simulink model "IEEE39_ClosedLoop_Native"  (R2025a)
settings: Solver=ode4  StartTime=0.0  StopTime=stopTime  FixedStep=dt  RelTol=1e-3
values from neighbouring files (symbols this model uses):
  dt = double(entry.step_s)    [run_fmu_cosim_sweep.m]    (also in run_ieee39_closed_loop.m; run_ieee39_native_closed_loop.m)
  loadStepTime = double(entry.load_step_s)    [run_ieee39_closed_loop.m]    (also in run_ieee39_native_closed_loop.m)
  stopTime = double(entry.stop_time_s)    [run_fmu_cosim_sweep.m]    (also in run_ieee39_closed_loop.m; run_ieee39_native_closed_loop.m; run_native_replay.m = simulateToTime)
settings Model: Creator=matthiasmees  LastModifiedBy=matthiasmees
settings DataIOCC: SaveOutput=off  SignalLogging=off  SaveTime=off

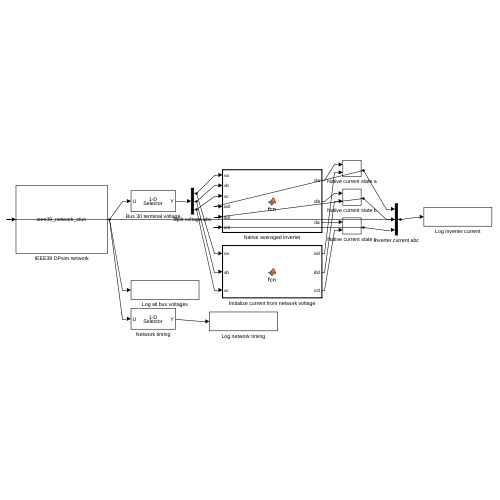
[thumbnail: Simulink's stored preview of the top-level diagram]
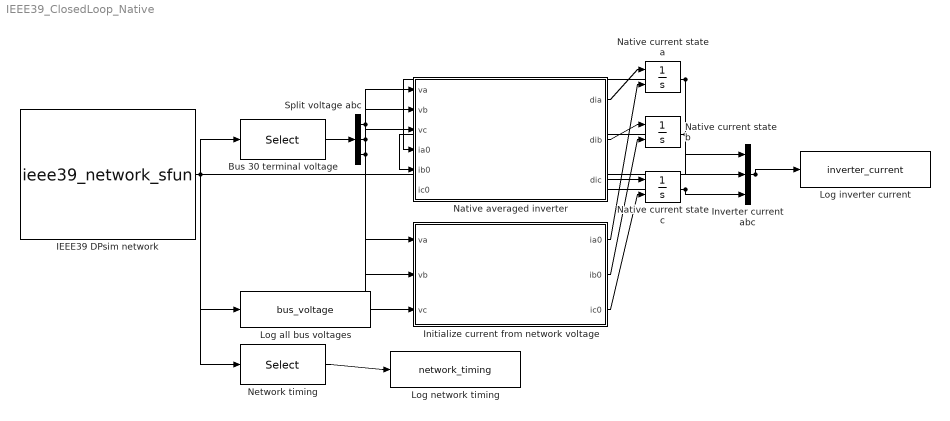
== system IEEE39_ClosedLoop_Native ==
  Bus 30 terminal voltage : Selector  InputPortWidth=119  IndexOptions=Index vector (dialog)  Indices=88:90  OutputSizes=1
  IEEE39 DPsim network : S-Function  FunctionName=ieee39_network_sfun  Parameters=dt,stopTime,loadStepTime  SFunctionDeploymentMode=off  EnableBusSupport=off
  Initialize current from network voltage : MATLAB Function  TreatAsAtomicUnit=on
  Inverter current abc : Mux  Inputs=3
  Log all bus voltages : ToWorkspace  VariableName=bus_voltage  SaveFormat=Timeseries  SampleTime=-1
  Log inverter current : ToWorkspace  VariableName=inverter_current  SaveFormat=Timeseries  SampleTime=-1
  Log network timing : ToWorkspace  VariableName=network_timing  SaveFormat=Timeseries  SampleTime=-1
  Native averaged inverter : MATLAB Function  TreatAsAtomicUnit=on
  Native current state a : Integrator  InitialConditionSource=external
  Native current state b : Integrator  InitialConditionSource=external
  Native current state c : Integrator  InitialConditionSource=external
  Network timing : Selector  InputPortWidth=119  IndexOptions=Index vector (dialog)  Indices=118:119  OutputSizes=1
  Split voltage abc : Demux  Outputs=3
  wires:
  IEEE39 DPsim network/1 -> Bus 30 terminal voltage/1, Log all bus voltages/1, Network timing/1
  Network timing/1 -> Log network timing/1
  Bus 30 terminal voltage/1 -> Split voltage abc/1
  Split voltage abc/1 -> Native averaged inverter/1(va), Initialize current from network voltage/1(va)
  Native current state a/1 -> Native averaged inverter/4(ia0), Inverter current abc/1
  Native averaged inverter/1(dia) -> Native current state a/1
  Initialize current from network voltage/1(ia0) -> Native current state a/2
  Split voltage abc/2 -> Native averaged inverter/2(vb), Initialize current from network voltage/2(vb)
  Native current state b/1 -> Native averaged inverter/5(ib0), Inverter current abc/2
  Native averaged inverter/2(dib) -> Native current state b/1
  Initialize current from network voltage/2(ib0) -> Native current state b/2
  Split voltage abc/3 -> Native averaged inverter/3(vc), Initialize current from network voltage/3(vc)
  Native current state c/1 -> Native averaged inverter/6(ic0), Inverter current abc/3
  Native averaged inverter/3(dic) -> Native current state c/1
  Initialize current from network voltage/3(ic0) -> Native current state c/2
  Inverter current abc/1 -> IEEE39 DPsim network/1, Log inverter current/1

== matlab function IEEE39_ClosedLoop_Native/Native averaged inverter ==
  data: va input; dia output; vb input; vc input; ia0 input; ib0 input; ic0 input; dib output; dic output
function [dia,dib,dic] = fcn(va,vb,vc,ia0,ib0,ic0)
%#codegen
P=125e6; Q=80.881e6; Vnom=345e3; Ipu=1.20; tau=5e-3;
a=(2/3)*(va-0.5*vb-0.5*vc);
b=(2/3)*(sqrt(3)/2)*(vb-vc); v2=a*a+b*b;
if v2<1, iaref=0; ibref=0; icref=0; else
 k=2/(3*v2); ialpha=k*(P*a+Q*b); ibeta=k*(P*b-Q*a);
 imax=Ipu*sqrt(2)*hypot(P,Q)/(sqrt(3)*Vnom); imag=hypot(ialpha,ibeta);
 if imag>imax, ialpha=ialpha*imax/imag; ibeta=ibeta*imax/imag; end
 iaref=ialpha; ibref=-0.5*ialpha+sqrt(3)/2*ibeta;
 icref=-0.5*ialpha-sqrt(3)/2*ibeta; end
 dia=(-iaref-ia0)/tau; dib=(-ibref-ib0)/tau; dic=(-icref-ic0)/tau;
end

== matlab function IEEE39_ClosedLoop_Native/Initialize current from network voltage ==
  data: va input; ia0 output; vb input; vc input; ib0 output; ic0 output
function [ia0,ib0,ic0] = fcn(va,vb,vc)
%#codegen
P=125e6; Q=80.881e6; Vnom=345e3; Ipu=1.20;
a=(2/3)*(va-0.5*vb-0.5*vc);
b=(2/3)*(sqrt(3)/2)*(vb-vc); v2=a*a+b*b;
if v2<1, ia0=0; ib0=0; ic0=0; else
 k=2/(3*v2); ialpha=k*(P*a+Q*b); ibeta=k*(P*b-Q*a);
 imax=Ipu*sqrt(2)*hypot(P,Q)/(sqrt(3)*Vnom); imag=hypot(ialpha,ibeta);
 if imag>imax, ialpha=ialpha*imax/imag; ibeta=ibeta*imax/imag; end
 ia0=-ialpha; ib0=0.5*ialpha-sqrt(3)/2*ibeta;
 ic0=0.5*ialpha+sqrt(3)/2*ibeta; end
end
